simulink model "WBR_Simulator"  (R2023b)
settings: Solver=FixedStepAuto  StartTime=0.0  StopTime=60  FixedStep=0.001  MaxStep=0.001
undefined symbols (not defined in the file or in its folder): DiscIntNeverNeededParam, magnitude, robot_stats, SIMPARAM, X, Y, Z
libraries: sm_lib x73, nesl_utility x50, simulink x17, slpidlib x6, dsparch4 x2
(part 6 of 7)

== system WBR_Simulator/腿建模/并联腿2 ==
  note: 出现过原始角速度跳变的情况
  note: 此处phi0为平行z轴为0,往越往x轴越大
  设定切向力矩 : Inport
  设定径向力 : Inport  Port=2
  Brick Solid : sm_lib/Body Elements/Brick Solid  GraphicAmbientColor=[0.15 0.15 0.15 1.0]  BasedOnType=Mass  BrickDimensions=[SIMPARAM.L5 0.01 0.01]  BrickDimensionsUnits=m  CenterOfMass=[0 0 0]  CenterOfMassUnits=m  GraphicDiffuseColor=[0.2 0.0 0.0]  Density=1000  DensityUnits=kg/m^3  DoExposeReferenceFrame=on  GraphicEmissiveColor=[0.0 0.0 0.0 1.0]  ExportEntireGeometry=on  SerializedFrames=<Frames><Frame><Id>Frame2</Id><Value><Name>A</Name><Origin><Source>GeometricFeature</Source><FeatureName>-x surface</FeatureName></Origin><PrimaryAxis><DefinedDirection>+Y</DefinedDirection><Source>ReferenceFrame</Source><SourceDirection>+Z</SourceDirection><FeatureName></FeatureName></PrimaryAxis><SecondaryAxis><DefinedDirection>+X</DefinedDirection><Source>ReferenceFrame</Source><SourceDirection>+X</SourceDirection><FeatureName></FeatureName></SecondaryAxis></Value></Frame><Frame><Id>Frame3</Id><Value><Name>E</Name><Origin><Source>GeometricFeature</Source><FeatureName>+x surface</FeatureName></Origin><PrimaryAxis><DefinedDirection>+Y</DefinedDirection><Source>ReferenceFrame</Source><SourceDirection>+Z</SourceDirection><FeatureName></FeatureName></PrimaryAxis><SecondaryAxis><DefinedDirection>+X</DefinedDirection><Source>ReferenceFrame</Source><SourceDirection>+X</SourceDirection><FeatureName></FeatureName></SecondaryAxis></Value></Frame></Frames>  MarkerShape=Sphere  MarkerSize=10  GraphicType=FromGeometry  InertiaType=CalculateFromGeometry  Mass=0.00001  MassUnits=kg  MomentsOfInertia=[1 1 1]  MomentsOfInertiaUnits=kg*m^2  GraphicOpacity=1.0  ProductsOfInertia=[0 0 0]  ProductsOfInertiaUnits=kg*m^2  GraphicShininess=75  GraphicSpecularColor=[0.5 0.5 0.5 1.0]  GraphicVisPropType=SimpleVisualProperties
  Brick Solid1 : sm_lib/Body Elements/Brick Solid  GraphicAmbientColor=[0.15 0.15 0.15 1.0]  BasedOnType=Mass  BrickDimensions="[robot_stats.length_thigh  0.01 0.01]"  BrickDimensionsUnits=m  CenterOfMass=[0 0 0]  CenterOfMassUnits=m  GraphicDiffuseColor=[0.0 0.8 1.0]  Density=1000  DensityUnits=kg/m^3  DoExposeReferenceFrame=off  GraphicEmissiveColor=[0.0 0.0 0.0 1.0]  ExportEntireGeometry=off  SerializedFrames=<Frames><Frame><Id>Frame1</Id><Value><Name>A</Name><Origin><Source>GeometricFeature</Source><FeatureName>-x surface</FeatureName></Origin><PrimaryAxis><DefinedDirection>+Y</DefinedDirection><Source>ReferenceFrame</Source><SourceDirection>+Z</SourceDirection><FeatureName></FeatureName></PrimaryAxis><SecondaryAxis><DefinedDirection>+X</DefinedDirection><Source>ReferenceFrame</Source><SourceDirection>+X</SourceDirection><FeatureName></FeatureName></SecondaryAxis></Value></Frame><Frame><Id>Frame2</Id><Value><Name>B</Name><Origin><Source>GeometricFeature</Source><FeatureName>+x surface</FeatureName></Origin><PrimaryAxis><DefinedDirection>-Y</DefinedDirection><Source>ReferenceFrame</Source><SourceDirection>+Z</SourceDirection><FeatureName></FeatureName></PrimaryAxis><SecondaryAxis><DefinedDirection>+X</DefinedDirection><Source>ReferenceFrame</Source><SourceDirection>+X</SourceDirection><FeatureName></FeatureName></SecondaryAxis></Value></Frame></Frames>  MarkerShape=Sphere  MarkerSize=10  GraphicType=FromGeometry  InertiaType=CalculateFromGeometry  Mass=robot_stats.mass_thigh_aver  MassUnits=kg  MomentsOfInertia=[1 1 1]  MomentsOfInertiaUnits=kg*m^2  GraphicOpacity=1.0  ProductsOfInertia=[0 0 0]  ProductsOfInertiaUnits=kg*m^2  GraphicShininess=75  GraphicSpecularColor=[0.5 0.5 0.5 1.0]  GraphicVisPropType=SimpleVisualProperties
  Brick Solid2 : sm_lib/Body Elements/Brick Solid  GraphicAmbientColor=[0.15 0.15 0.15 1.0]  BasedOnType=Mass  BrickDimensions="[robot_stats.length_thigh  0.01 0.01]"  BrickDimensionsUnits=m  CenterOfMass=[0 0 0]  CenterOfMassUnits=m  GraphicDiffuseColor=[0.0 0.8 1.0]  Density=1000  DensityUnits=kg/m^3  DoExposeReferenceFrame=off  GraphicEmissiveColor=[0.0 0.0 0.0 1.0]  ExportEntireGeometry=off  SerializedFrames=<Frames><Frame><Id>Frame1</Id><Value><Name>E</Name><Origin><Source>GeometricFeature</Source><FeatureName>-x surface</FeatureName></Origin><PrimaryAxis><DefinedDirection>-Y</DefinedDirection><Source>ReferenceFrame</Source><SourceDirection>+Z</SourceDirection><FeatureName></FeatureName></PrimaryAxis><SecondaryAxis><DefinedDirection>+X</DefinedDirection><Source>ReferenceFrame</Source><SourceDirection>+X</SourceDirection><FeatureName></FeatureName></SecondaryAxis></Value></Frame><Frame><Id>Frame2</Id><Value><Name>D</Name><Origin><Source>GeometricFeature</Source><FeatureName>+x surface</FeatureName></Origin><PrimaryAxis><DefinedDirection>+Y</DefinedDirection><Source>ReferenceFrame</Source><SourceDirection>+Z</SourceDirection><FeatureName></FeatureName></PrimaryAxis><SecondaryAxis><DefinedDirection>+X</DefinedDirection><Source>ReferenceFrame</Source><SourceDirection>+X</SourceDirection><FeatureName></FeatureName></SecondaryAxis></Value></Frame></Frames>  MarkerShape=Sphere  MarkerSize=10  GraphicType=FromGeometry  InertiaType=CalculateFromGeometry  Mass=robot_stats.mass_thigh_aver  MassUnits=kg  MomentsOfInertia=[1 1 1]  MomentsOfInertiaUnits=kg*m^2  GraphicOpacity=1.0  ProductsOfInertia=[0 0 0]  ProductsOfInertiaUnits=kg*m^2  GraphicShininess=75  GraphicSpecularColor=[0.5 0.5 0.5 1.0]  GraphicVisPropType=SimpleVisualProperties
  Brick Solid3 : sm_lib/Body Elements/Brick Solid  GraphicAmbientColor=[0.15 0.15 0.15 1.0]  BasedOnType=Mass  BrickDimensions="[robot_stats.length_calf  0.01 0.01]"  BrickDimensionsUnits=m  CenterOfMass=[0 0 0]  CenterOfMassUnits=m  GraphicDiffuseColor=[1.0 0.0 0.0]  Density=1000  DensityUnits=kg/m^3  DoExposeReferenceFrame=off  GraphicEmissiveColor=[0.0 0.0 0.0 1.0]  ExportEntireGeometry=off  SerializedFrames=<Frames><Frame><Id>Frame1</Id><Value><Name>B</Name><Origin><Source>GeometricFeature</Source><FeatureName>-x surface</FeatureName></Origin><PrimaryAxis><DefinedDirection>-Y</DefinedDirection><Source>ReferenceFrame</Source><SourceDirection>+Z</SourceDirection><FeatureName></FeatureName></PrimaryAxis><SecondaryAxis><DefinedDirection>+X</DefinedDirection><Source>ReferenceFrame</Source><SourceDirection>+X</SourceDirection><FeatureName></FeatureName></SecondaryAxis></Value></Frame><Frame><Id>Frame2</Id><Value><Name>C</Name><Origin><Source>GeometricFeature</Source><FeatureName>+x surface</FeatureName></Origin><PrimaryAxis><DefinedDirection>-Y</DefinedDirection><Source>ReferenceFrame</Source><SourceDirection>+Z</SourceDirection><FeatureName></FeatureName></PrimaryAxis><SecondaryAxis><DefinedDirection>+X</DefinedDirection><Source>ReferenceFrame</Source><SourceDirection>+X</SourceDirection><FeatureName></FeatureName></SecondaryAxis></Value></Frame></Frames>  MarkerShape=Sphere  MarkerSize=10  GraphicType=FromGeometry  InertiaType=CalculateFromGeometry  Mass=robot_stats.mass_calf_aver  MassUnits=kg  MomentsOfInertia=[1 1 1]  MomentsOfInertiaUnits=kg*m^2  GraphicOpacity=1.0  ProductsOfInertia=[0 0 0]  ProductsOfInertiaUnits=kg*m^2  GraphicShininess=75  GraphicSpecularColor=[0.5 0.5 0.5 1.0]  GraphicVisPropType=SimpleVisualProperties
  Brick Solid4 : sm_lib/Body Elements/Brick Solid  GraphicAmbientColor=[0.15 0.15 0.15 1.0]  BasedOnType=Mass  BrickDimensions="[robot_stats.length_calf  0.01 0.01]"  BrickDimensionsUnits=m  CenterOfMass=[0 0 0]  CenterOfMassUnits=m  GraphicDiffuseColor=[1.0 0.0 0.0]  Density=1000  DensityUnits=kg/m^3  DoExposeReferenceFrame=off  GraphicEmissiveColor=[0.0 0.0 0.0 1.0]  ExportEntireGeometry=off  SerializedFrames=<Frames><Frame><Id>Frame1</Id><Value><Name>C</Name><Origin><Source>GeometricFeature</Source><FeatureName>-x surface</FeatureName></Origin><PrimaryAxis><DefinedDirection>-Y</DefinedDirection><Source>ReferenceFrame</Source><SourceDirection>+Z</SourceDirection><FeatureName></FeatureName></PrimaryAxis><SecondaryAxis><DefinedDirection>+X</DefinedDirection><Source>ReferenceFrame</Source><SourceDirection>+X</SourceDirection><FeatureName></FeatureName></SecondaryAxis></Value></Frame><Frame><Id>Frame2</Id><Value><Name>D</Name><Origin><Source>GeometricFeature</Source><FeatureName>+x surface</FeatureName></Origin><PrimaryAxis><DefinedDirection>-Y</DefinedDirection><Source>ReferenceFrame</Source><SourceDirection>+Z</SourceDirection><FeatureName></FeatureName></PrimaryAxis><SecondaryAxis><DefinedDirection>+X</DefinedDirection><Source>ReferenceFrame</Source><SourceDirection>+X</SourceDirection><FeatureName></FeatureName></SecondaryAxis></Value></Frame></Frames>  MarkerShape=Sphere  MarkerSize=10  GraphicType=FromGeometry  InertiaType=CalculateFromGeometry  Mass=robot_stats.mass_calf_aver  MassUnits=kg  MomentsOfInertia=[1 1 1]  MomentsOfInertiaUnits=kg*m^2  GraphicOpacity=1.0  ProductsOfInertia=[0 0 0]  ProductsOfInertiaUnits=kg*m^2  GraphicShininess=75  GraphicSpecularColor=[0.5 0.5 0.5 1.0]  GraphicVisPropType=SimpleVisualProperties
  Brick Solid5 : sm_lib/Body Elements/Brick Solid  GraphicAmbientColor=[0.15 0.15 0.15 1.0]  BasedOnType=Mass  BrickDimensions=[0.01 0.01 0.01]  BrickDimensionsUnits=m  CenterOfMass=[0 0 0]  CenterOfMassUnits=m  GraphicDiffuseColor=[0.5 0.5 0.5]  Density=1000  DensityUnits=kg/m^3  DoExposeReferenceFrame=on  GraphicEmissiveColor=[0.0 0.0 0.0 1.0]  ExportEntireGeometry=off  SerializedFrames=<Frames><Frame><Id>Frame1</Id><Value><Name>joint</Name><Origin><Source>CenterOfMassFrame</Source><FeatureName></FeatureName></Origin><PrimaryAxis><DefinedDirection>-Z</DefinedDirection><Source>ReferenceFrame</Source><SourceDirection>+Z</SourceDirection><FeatureName></FeatureName></PrimaryAxis><SecondaryAxis><DefinedDirection>+X</DefinedDirection><Source>ReferenceFrame</Source><SourceDirection>+X</SourceDirection><FeatureName></FeatureName></SecondaryAxis></Value></Frame></Frames>  MarkerShape=Sphere  MarkerSize=10  GraphicType=FromGeometry  InertiaType=CalculateFromGeometry  Mass=0.00001  MassUnits=kg  MomentsOfInertia=[1 1 1]  MomentsOfInertiaUnits=kg*m^2  GraphicOpacity=1.0  ProductsOfInertia=[0 0 0]  ProductsOfInertiaUnits=kg*m^2  GraphicShininess=75  GraphicSpecularColor=[0.5 0.5 0.5 1.0]  GraphicVisPropType=SimpleVisualProperties
  Bus Creator : BusCreator  Inputs=4
  Bus Creator1 : BusCreator  Inputs=2
  Bus Creator2 : BusCreator  Inputs=2
  Bus Creator5 : BusCreator  Inputs=2
  Bus Creator6 : BusCreator  Inputs=4
  Bus Selector : BusSelector  OutputSignals=phi_1,phi_4
  Bus Selector1 : BusSelector  OutputSignals=signal2.phi_1,signal2.phi_4,signal2.wphi_1,signal2.wphi_4,signal1.phi_2,signal1.phi_3
  Bus Selector2 : BusSelector  OutputSignals=signal2.phi_1,signal1.phi_2,signal1.phi_3,signal2.phi_4,signal2.wphi_1,signal2.wphi_4
  Connection Label1 : ConnectionLabel  Label=base_frame
  Connection Label6 : ConnectionLabel  Label=base_frame
  PS-Simulink Converter{,1..3} (4 alike) : nesl_utility/PS-Simulink Converter  PhysicalDomain=network_engine_domain  SubClassName=ps_output  LeftPortType=input  RightPortType=output  PseudoPeriodic=off  Frequencies=[]  VectorFormat=1-D array  Unit=inherit  AffineConversion=off
  Revolute Joint : sm_lib/Joints/Revolute Joint  JointMode=Normal  SenseConstraintForce=off  SenseConstraintForceX=off  SenseConstraintForceY=off  SenseConstraintForceZ=off  SenseConstraintTorque=off  SenseConstraintTorqueX=off  SenseConstraintTorqueY=off  SenseConstraintTorqueZ=off  SenseTotalForce=off  SenseTotalForceX=off  SenseTotalForceY=off  SenseTotalForceZ=off  SenseTotalTorque=off  SenseTotalTorqueX=off  SenseTotalTorqueY=off  SenseTotalTorqueZ=off  CompositeWrenchDir=FollowerOnBase  CompositeWrenchFrame=BaseFrame  EquilibriumPosition=0  EquilibriumPositionUnits=deg  SpringStiffness=0  SpringStiffnessUnits=N*m/deg  DampingCoefficient=0  DampingCoefficientUnits=N*m/(deg/s)  TorqueActuationMode=InputTorque  MotionActuationMode=ComputedMotion  SensePosition=on  SenseVelocity=on  SenseAcceleration=off  SenseTorqueForce=off  SenseLowerLimitTorqueForce=off  SenseUpperLimitTorqueForce=off  LowerLimitSpecify=off  LowerLimitBound=-90  LowerLimitBoundUnits=deg  LowerLimitStiffness=1e4  LowerLimitStiffnessUnits=N*m/deg  LowerLimitDamping=10  LowerLimitDampingUnits=N*m/(deg/s)  LowerLimitTransitionRegionWidth=0.1  LowerLimitTransitionRegionWidthUnits=deg  UpperLimitSpecify=off  UpperLimitBound=90  UpperLimitBoundUnits=deg  UpperLimitStiffness=1e4  UpperLimitStiffnessUnits=N*m/deg  UpperLimitDamping=10  UpperLimitDampingUnits=N*m/(deg/s)  UpperLimitTransitionRegionWidth=0.1  UpperLimitTransitionRegionWidthUnits=deg  PositionTargetSpecify=on  PositionTargetPriority=High  PositionTargetValue=SIMPARAM.init_phi1  PositionTargetValueUnits=rad  VelocityTargetSpecify=off  VelocityTargetPriority=High  VelocityTargetValue=0  VelocityTargetValueUnits=deg/s
  Revolute Joint1 : sm_lib/Joints/Revolute Joint  JointMode=Normal  SenseConstraintForce=off  SenseConstraintForceX=off  SenseConstraintForceY=off  SenseConstraintForceZ=off  SenseConstraintTorque=off  SenseConstraintTorqueX=off  SenseConstraintTorqueY=off  SenseConstraintTorqueZ=off  SenseTotalForce=off  SenseTotalForceX=off  SenseTotalForceY=off  SenseTotalForceZ=off  SenseTotalTorque=off  SenseTotalTorqueX=off  SenseTotalTorqueY=off  SenseTotalTorqueZ=off  CompositeWrenchDir=FollowerOnBase  CompositeWrenchFrame=BaseFrame  EquilibriumPosition=0  EquilibriumPositionUnits=deg  SpringStiffness=0  SpringStiffnessUnits=N*m/deg  DampingCoefficient=0  DampingCoefficientUnits=N*m/(deg/s)  TorqueActuationMode=InputTorque  MotionActuationMode=ComputedMotion  SensePosition=on  SenseVelocity=on  SenseAcceleration=off  SenseTorqueForce=off  SenseLowerLimitTorqueForce=off  SenseUpperLimitTorqueForce=off  LowerLimitSpecify=off  LowerLimitBound=-90  LowerLimitBoundUnits=deg  LowerLimitStiffness=1e4  LowerLimitStiffnessUnits=N*m/deg  LowerLimitDamping=10  LowerLimitDampingUnits=N*m/(deg/s)  LowerLimitTransitionRegionWidth=0.1  LowerLimitTransitionRegionWidthUnits=deg  UpperLimitSpecify=off  UpperLimitBound=90  UpperLimitBoundUnits=deg  UpperLimitStiffness=1e4  UpperLimitStiffnessUnits=N*m/deg  UpperLimitDamping=10  UpperLimitDampingUnits=N*m/(deg/s)  UpperLimitTransitionRegionWidth=0.1  UpperLimitTransitionRegionWidthUnits=deg  PositionTargetSpecify=on  PositionTargetPriority=High  PositionTargetValue=SIMPARAM.init_phi4  PositionTargetValueUnits=rad  VelocityTargetSpecify=off  VelocityTargetPriority=High  VelocityTargetValue=0  VelocityTargetValueUnits=deg/s
  Revolute Joint2 : sm_lib/Joints/Revolute Joint  JointMode=Normal  SenseConstraintForce=off  SenseConstraintForceX=off  SenseConstraintForceY=off  SenseConstraintForceZ=off  SenseConstraintTorque=off  SenseConstraintTorqueX=off  SenseConstraintTorqueY=off  SenseConstraintTorqueZ=off  SenseTotalForce=off  SenseTotalForceX=off  SenseTotalForceY=off  SenseTotalForceZ=off  SenseTotalTorque=off  SenseTotalTorqueX=off  SenseTotalTorqueY=off  SenseTotalTorqueZ=off  CompositeWrenchDir=FollowerOnBase  CompositeWrenchFrame=BaseFrame  EquilibriumPosition=0  EquilibriumPositionUnits=deg  SpringStiffness=0  SpringStiffnessUnits=N*m/deg  DampingCoefficient=0  DampingCoefficientUnits=N*m/(deg/s)  TorqueActuationMode=NoTorque  MotionActuationMode=ComputedMotion  SensePosition=off  SenseVelocity=off  SenseAcceleration=off  SenseTorqueForce=off  SenseLowerLimitTorqueForce=off  SenseUpperLimitTorqueForce=off  LowerLimitSpecify=off  LowerLimitBound=-90  LowerLimitBoundUnits=deg  LowerLimitStiffness=1e4  LowerLimitStiffnessUnits=N*m/deg  LowerLimitDamping=10  LowerLimitDampingUnits=N*m/(deg/s)  LowerLimitTransitionRegionWidth=0.1  LowerLimitTransitionRegionWidthUnits=deg  UpperLimitSpecify=off  UpperLimitBound=90  UpperLimitBoundUnits=deg  UpperLimitStiffness=1e4  UpperLimitStiffnessUnits=N*m/deg  UpperLimitDamping=10  UpperLimitDampingUnits=N*m/(deg/s)  UpperLimitTransitionRegionWidth=0.1  UpperLimitTransitionRegionWidthUnits=deg  PositionTargetSpecify=on  PositionTargetPriority=High  PositionTargetValue=SIMPARAM.init_phi1-SIMPARAM.init_phi2  PositionTargetValueUnits=rad  VelocityTargetSpecify=off  VelocityTargetPriority=High  VelocityTargetValue=0  VelocityTargetValueUnits=deg/s
  Revolute Joint3 : sm_lib/Joints/Revolute Joint  JointMode=Normal  SenseConstraintForce=off  SenseConstraintForceX=off  SenseConstraintForceY=off  SenseConstraintForceZ=off  SenseConstraintTorque=off  SenseConstraintTorqueX=off  SenseConstraintTorqueY=off  SenseConstraintTorqueZ=off  SenseTotalForce=off  SenseTotalForceX=off  SenseTotalForceY=off  SenseTotalForceZ=off  SenseTotalTorque=off  SenseTotalTorqueX=off  SenseTotalTorqueY=off  SenseTotalTorqueZ=off  CompositeWrenchDir=FollowerOnBase  CompositeWrenchFrame=BaseFrame  EquilibriumPosition=0  EquilibriumPositionUnits=deg  SpringStiffness=0  SpringStiffnessUnits=N*m/deg  DampingCoefficient=0  DampingCoefficientUnits=N*m/(deg/s)  TorqueActuationMode=NoTorque  MotionActuationMode=ComputedMotion  SensePosition=off  SenseVelocity=off  SenseAcceleration=off  SenseTorqueForce=off  SenseLowerLimitTorqueForce=off  SenseUpperLimitTorqueForce=off  LowerLimitSpecify=off  LowerLimitBound=-90  LowerLimitBoundUnits=deg  LowerLimitStiffness=1e4  LowerLimitStiffnessUnits=N*m/deg  LowerLimitDamping=10  LowerLimitDampingUnits=N*m/(deg/s)  LowerLimitTransitionRegionWidth=0.1  LowerLimitTransitionRegionWidthUnits=deg  UpperLimitSpecify=off  UpperLimitBound=90  UpperLimitBoundUnits=deg  UpperLimitStiffness=1e4  UpperLimitStiffnessUnits=N*m/deg  UpperLimitDamping=10  UpperLimitDampingUnits=N*m/(deg/s)  UpperLimitTransitionRegionWidth=0.1  UpperLimitTransitionRegionWidthUnits=deg  PositionTargetSpecify=on  PositionTargetPriority=High  PositionTargetValue=pi-(SIMPARAM.init_phi3-SIMPARAM.init_phi4)  PositionTargetValueUnits=rad  VelocityTargetSpecify=off  VelocityTargetPriority=High  VelocityTargetValue=0  VelocityTargetValueUnits=deg/s
  Revolute Joint5 : sm_lib/Joints/Revolute Joint  JointMode=Normal  SenseConstraintForce=off  SenseConstraintForceX=off  SenseConstraintForceY=off  SenseConstraintForceZ=off  SenseConstraintTorque=off  SenseConstraintTorqueX=off  SenseConstraintTorqueY=off  SenseConstraintTorqueZ=off  SenseTotalForce=off  SenseTotalForceX=off  SenseTotalForceY=off  SenseTotalForceZ=off  SenseTotalTorque=off  SenseTotalTorqueX=off  SenseTotalTorqueY=off  SenseTotalTorqueZ=off  CompositeWrenchDir=FollowerOnBase  CompositeWrenchFrame=BaseFrame  EquilibriumPosition=0  EquilibriumPositionUnits=deg  SpringStiffness=0  SpringStiffnessUnits=N*m/deg  DampingCoefficient=0  DampingCoefficientUnits=N*m/(deg/s)  TorqueActuationMode=NoTorque  MotionActuationMode=ComputedMotion  SensePosition=off  SenseVelocity=off  SenseAcceleration=off  SenseTorqueForce=off  SenseLowerLimitTorqueForce=off  SenseUpperLimitTorqueForce=off  LowerLimitSpecify=off  LowerLimitBound=-90  LowerLimitBoundUnits=deg  LowerLimitStiffness=1e4  LowerLimitStiffnessUnits=N*m/deg  LowerLimitDamping=10  LowerLimitDampingUnits=N*m/(deg/s)  LowerLimitTransitionRegionWidth=0.1  LowerLimitTransitionRegionWidthUnits=deg  UpperLimitSpecify=off  UpperLimitBound=90  UpperLimitBoundUnits=deg  UpperLimitStiffness=1e4  UpperLimitStiffnessUnits=N*m/deg  UpperLimitDamping=10  UpperLimitDampingUnits=N*m/(deg/s)  UpperLimitTransitionRegionWidth=0.1  UpperLimitTransitionRegionWidthUnits=deg  PositionTargetSpecify=off  PositionTargetPriority=High  PositionTargetValue=0  PositionTargetValueUnits=deg  VelocityTargetSpecify=off  VelocityTargetPriority=High  VelocityTargetValue=0  VelocityTargetValueUnits=deg/s
  Simulink-PS Converter : nesl_utility/Simulink-PS Converter  PhysicalDomain=network_engine_domain  SubClassName=ps_input  LeftPortType=input  RightPortType=output  PseudoPeriodic=off  Frequencies=[]  NoiseDistribution=none  NoiseParameters=[]  Unit=1  AffineConversion=off  FilteringAndDerivatives=provide  SimscapeFilterOrder=1  InputFilterTimeConstant=0.001  UdotUserProvided=0
  Simulink-PS Converter1 : nesl_utility/Simulink-PS Converter  PhysicalDomain=network_engine_domain  SubClassName=ps_input  LeftPortType=input  RightPortType=output  PseudoPeriodic=off  Frequencies=[]  NoiseDistribution=none  NoiseParameters=[]  Unit=1  AffineConversion=off  FilteringAndDerivatives=provide  SimscapeFilterOrder=1  InputFilterTimeConstant=0.001  UdotUserProvided=0
  Spatial Contact Force2 : sm_lib/Forces and Torques/Spatial Contact Force  SenseContactBaseRotation=off  SenseContactBaseTranslation=off  CoefficientOfDynamicFriction=0.3  CoefficientOfStaticFriction=0.5  NormalDamping=1e6  NormalDampingUnits=N/(m/s)  SenseContactSignal=off  NormalStiffness=1e6  NormalStiffnessUnits=N/m  FrictionalCriticalVelocity=1e-3  FrictionalCriticalVelocityUnits=m/s  ZeroCrossDetectContactStartAndEnd=off  SenseContactFollowerRotation=off  SenseContactFollowerTranslation=off  FrictionType=SmoothStickSlip  SenseFrictionalForceMagnitude=off  SenseNormalForceMagnitude=off  NormalForceType=SmoothSpringDamper  SenseNormalVelocity=off  SensePenetrationDepth=off  SenseSeparationDistance=off  SenseTangentialVelocity=off  NormalTransitionRegionWidth=1e-4  NormalTransitionRegionWidthUnits=m
  Spatial Contact Force7 : sm_lib/Forces and Torques/Spatial Contact Force  SenseContactBaseRotation=off  SenseContactBaseTranslation=off  CoefficientOfDynamicFriction=0.3  CoefficientOfStaticFriction=0.5  NormalDamping=1e6  NormalDampingUnits=N/(m/s)  SenseContactSignal=off  NormalStiffness=1e6  NormalStiffnessUnits=N/m  FrictionalCriticalVelocity=1e-3  FrictionalCriticalVelocityUnits=m/s  ZeroCrossDetectContactStartAndEnd=off  SenseContactFollowerRotation=off  SenseContactFollowerTranslation=off  FrictionType=SmoothStickSlip  SenseFrictionalForceMagnitude=off  SenseNormalForceMagnitude=off  NormalForceType=SmoothSpringDamper  SenseNormalVelocity=off  SensePenetrationDepth=off  SenseSeparationDistance=off  SenseTangentialVelocity=off  NormalTransitionRegionWidth=1e-4  NormalTransitionRegionWidthUnits=m
  Zero-Order Hold{,1..3} (4 alike) : ZeroOrderHold  SampleTime=0.001
  五连杆正解算矩阵(关节转至末端) : Subsystem
  腿末端控制器 : Subsystem
  解算phi2&phi3_1 : Subsystem
  运动学解算验证(仅可证明旋转矩阵 : Subsystem
  基坐标 : PMIOPort  Side=Left
  轮毂坐标轴 : PMIOPort  Port=2  Side=Left
  底盘地面碰撞 : PMIOPort  Port=3  Side=Right
  底盘飞坡碰撞 : PMIOPort  Port=4  Side=Right
  phi_0 : Outport
  L_0 : Outport  Port=2
  real_vq : Outport  Port=3
  real_vd : Outport  Port=4
  valid_tqd : Outport  Port=5
  wires:
  Bus Creator2/1 -> Bus Selector2/1, Bus Selector1/1  "腿关节角度集"
  腿末端控制器/3(R) -> [R]
  Bus Selector1/2 -> 五连杆正解算矩阵(关节转至末端)/2(phi_4)  "<phi_4>"
  Bus Creator/1 -> Bus Creator2/2, Bus Selector/1
  Bus Selector1/6 -> 五连杆正解算矩阵(关节转至末端)/6(phi_3)  "<phi_3>"
  五连杆正解算矩阵(关节转至末端)/1(J) -> 腿末端控制器/6(J)  "J矩阵"
  Bus Selector/1 -> 解算phi2&phi3_1/1(phi1)  "<phi_1>"
  Bus Selector2/2 -> Bus Creator6/2  "<phi_2>"
  Bus Selector/2 -> 解算phi2&phi3_1/2(phi4)  "<phi_4>"
  腿末端控制器/4(R_inv) -> [R_inv]
  Bus Selector1/4 -> 五连杆正解算矩阵(关节转至末端)/4(wphi_4)  "<wphi_4>"
  Bus Selector1/3 -> 五连杆正解算矩阵(关节转至末端)/3(wphi_1)  "<wphi_1>"
  Bus Selector1/5 -> 五连杆正解算矩阵(关节转至末端)/5(phi_2)  "<phi_2>"
  Bus Selector2/5 -> 腿末端控制器/2(wphi_1)  "<wphi_1>"
  Bus Selector2/6 -> 腿末端控制器/3(wphi_4)  "<wphi_4>"
  Bus Selector1/1 -> 五连杆正解算矩阵(关节转至末端)/1(phi_1)  "<phi_1>"
  [R_inv] -> 运动学解算验证(仅可证明旋转矩阵/2(R_inv)
  [R] -> 运动学解算验证(仅可证明旋转矩阵/1(R)
  Bus Creator1/1 -> ?  "关节扭矩"
  腿末端控制器/5(phi_0) -> phi_0/1
  腿末端控制器/6(L_0) -> L_0/1
  腿末端控制器/8(real_vd) -> real_vd/1
  腿末端控制器/7(real_vq) -> real_vq/1
  设定切向力矩/1 -> 腿末端控制器/4(set_tq)
  设定径向力/1 -> 腿末端控制器/5(set_fd)
  PS-Simulink Converter/1 -> Zero-Order Hold/1
  PS-Simulink Converter1/1 -> Zero-Order Hold1/1
  腿末端控制器/1(torque_1) -> Bus Creator1/1, Simulink-PS Converter/1
  腿末端控制器/2(torque_4) -> Bus Creator1/2, Simulink-PS Converter1/1
  PS-Simulink Converter2/1 -> Zero-Order Hold2/1
  PS-Simulink Converter3/1 -> Zero-Order Hold3/1
  腿末端控制器/9(valid_tqd) -> valid_tqd/1
  解算phi2&phi3_1/1(phi2) -> Bus Creator5/1  "phi_2"
  解算phi2&phi3_1/2(phi3) -> Bus Creator5/2  "phi_3"
  Bus Creator5/1 -> Bus Creator2/1
  Bus Selector2/1 -> Bus Creator6/1  "<phi_1>"
  Bus Selector2/4 -> Bus Creator6/4  "<phi_4>"
  Bus Selector2/3 -> Bus Creator6/3  "<phi_3>"
  Bus Creator6/1 -> 腿末端控制器/1(phi)
  Zero-Order Hold/1 -> Bus Creator/1  "phi_1"
  Zero-Order Hold1/1 -> Bus Creator/2  "phi_4"
  Zero-Order Hold2/1 -> Bus Creator/3  "wphi_1"
  Zero-Order Hold3/1 -> Bus Creator/4  "wphi_4"
  connections:
  Brick Solid/LConn2 -- Revolute Joint1/LConn1
  Revolute Joint2/RConn1 -- Brick Solid3/LConn1
  PS-Simulink Converter1/LConn1 -- Revolute Joint1/RConn2
  Revolute Joint/LConn1 -- Brick Solid/LConn1
  Revolute Joint/RConn2 -- PS-Simulink Converter/LConn1
  Brick Solid4/RConn1 -- Revolute Joint3/RConn1
  Revolute Joint/RConn1 -- Brick Solid1/LConn1
  Brick Solid4/LConn1 -- Revolute Joint5/LConn1
  Brick Solid5/RConn1 -- Brick Solid3/RConn1 -- Revolute Joint5/RConn1 -- 运动学解算验证(仅可证明旋转矩阵/RConn1
  Revolute Joint/RConn3 -- PS-Simulink Converter2/LConn1
  Connection Label6/LConn1 -- 运动学解算验证(仅可证明旋转矩阵/LConn1
  Revolute Joint1/RConn3 -- PS-Simulink Converter3/LConn1
  Brick Solid2/RConn1 -- Revolute Joint3/LConn1
  基坐标/RConn1 -- Connection Label1/LConn1 -- Brick Solid/RConn1
  Revolute Joint/LConn2 -- Simulink-PS Converter/RConn1
  Simulink-PS Converter1/RConn1 -- Revolute Joint1/LConn2
  Revolute Joint1/RConn1 -- Brick Solid2/LConn1
  Brick Solid5/LConn1 -- 轮毂坐标轴/RConn1
  Brick Solid1/RConn1 -- Revolute Joint2/LConn1
  Spatial Contact Force2/LConn1 -- 底盘地面碰撞/RConn1
  Spatial Contact Force7/RConn1 -- Brick Solid/RConn2 -- Spatial Contact Force2/RConn1
  Spatial Contact Force7/LConn1 -- 底盘飞坡碰撞/RConn1

== system WBR_Simulator/腿建模/串联腿/五连杆正解算矩阵(关节转至末端) ==
  phi_1 : Inport
  phi_2 : Inport  Port=2
  Add : Sum  Inputs=-+
  Add1 : Sum  Inputs=-+
  Add2 : Sum  Inputs=+-
  Add3 : Sum  Inputs=+-
  Constant : Constant  Value=SIMPARAM.L2
  Constant1 : Constant  Value=SIMPARAM.L2
  Constant{2,4..5,7} (4 alike) : Constant  Value=0
  Constant3 : Constant  Value=SIMPARAM.L1
  Constant8 : Constant  Value=SIMPARAM.L1
  Divide{,1..3} (4 alike) : Product  Inputs=**
  MATLAB Function : MATLAB Function  TreatAsAtomicUnit=on
  Sin1 : Trigonometry
  Sin2 : Trigonometry
  Sin3 : Trigonometry  Operator=cos
  Sin4 : Trigonometry  Operator=cos
  J : Outport
  wires:
  phi_1/1 -> [phi_1]
  phi_2/1 -> [phi_2]
  [phi_1] -> Sin1/1
  MATLAB Function/1(J) -> J/1
  Constant4/1 -> Add/2
  Sin1/1 -> Add/1
  Constant8/1 -> Divide/2
  Add/1 -> Divide/1
  Add1/1 -> Divide1/1
  Sin2/1 -> Add1/1
  Constant2/1 -> Add1/2
  [phi_2] -> Sin2/1
  Constant/1 -> Divide1/2
  Add2/1 -> Divide2/1
  Sin3/1 -> Add2/1
  Constant5/1 -> Add2/2
  [phi_1] -> Sin3/1
  Constant3/1 -> Divide2/2
  Constant1/1 -> Divide3/2
  Constant7/1 -> Add3/2
  Add3/1 -> Divide3/1
  [phi_2] -> Sin4/1
  Sin4/1 -> Add3/1
  Divide/1 -> MATLAB Function/1(J11)
  Divide1/1 -> MATLAB Function/2(J12)
  Divide2/1 -> MATLAB Function/3(J21)
  Divide3/1 -> MATLAB Function/4(J22)

== system WBR_Simulator/腿建模/串联腿/腿末端控制器 ==
  phi : Inport
  wphi_1 : Inport  Port=2
  wphi_2 : Inport  Port=3
  set_tq : Inport  Port=4
  set_fd : Inport  Port=5
  J : Inport  Port=6
  Bus Selector : BusSelector  OutputSignals=phi_1,phi_2
  Constant : Constant  Value=0
  Constant1 : Constant
  Constant2 : Constant
  Constant3 : Constant  Value=0
  Divide : Product  Inputs=*/
  From2 : From  Commented=on  GotoTag=real_vxy
  From5 : From  Commented=on  GotoTag=J
  Mux : Mux  Inputs=2
  Mux1 : Mux
  Product : Product  Inputs=/  Multiplication=Matrix(*)
  Product8 : Product  Multiplication=Matrix(*)
  Reshape : Reshape  OutputDimensionality=Customize  OutputDimensions=[2,2]
  xy运动 : Subsystem  Commented=on
  极坐标运动控制器 : Subsystem
  笛卡尔坐标系转极坐标系 : Subsystem
  torque_1 : Outport
  torque_2 : Outport  Port=2
  R : Outport  Port=3
  R_inv : Outport  Port=4
  phi_0 : Outport  Port=5
  L_0 : Outport  Port=6
  real_vq : Outport  Port=7
  real_vd : Outport  Port=8
  valid_tqd : Outport  Port=9
  wires:
  J/1 -> [J]
  wphi_1/1 -> [wphi_1]
  wphi_2/1 -> [wphi_2]
  Product8/1 -> [real_vxy]
  [wphi_2] -> Mux/2
  [J] -> Product8/1
  Mux/1 -> Product8/2
  [wphi_1] -> Mux/1
  From2/1 -> xy运动/1(real_vxy)
  [real_vxy] -> 极坐标运动控制器/1(real_vxy)
  [R] -> 极坐标运动控制器/2(R)
  [J] -> 极坐标运动控制器/3(J)
  From5/1 -> xy运动/2(J)
  笛卡尔坐标系转极坐标系/1(R) -> [R], R/1, Product/1
  Product/1 -> R_inv/1
  极坐标运动控制器/2(torque_2) -> torque_2/1
  极坐标运动控制器/1(torque_1) -> torque_1/1
  笛卡尔坐标系转极坐标系/3(L_0) -> [L_0], L_0/1
  笛卡尔坐标系转极坐标系/2(phi_0) -> phi_0/1
  set_tq/1 -> 极坐标运动控制器/6(set_tq)
  set_fd/1 -> 极坐标运动控制器/7(set_fd)
  极坐标运动控制器/4(real_vd) -> real_vd/1
  极坐标运动控制器/3(real_vq) -> real_vq/1
  [phi_2] -> 笛卡尔坐标系转极坐标系/2(phi_2)
  [phi_1] -> 笛卡尔坐标系转极坐标系/1(phi_1)
  Mux1/1 -> Reshape/1
  [L_0] -> Divide/2
  Constant1/1 -> Mux1/4  "M22"
  Reshape/1 -> [M]
  [M] -> 极坐标运动控制器/4(M)
  Constant/1 -> Mux1/3  "M12"
  Constant3/1 -> Mux1/2  "M21"
  Constant2/1 -> Divide/1
  Divide/1 -> Mux1/1  "M11"
  极坐标运动控制器/5(valid_tqd) -> valid_tqd/1
  [phi] -> 极坐标运动控制器/5(In5)
  Bus Selector/1 -> [phi_1]  "<phi_1>"
  Bus Selector/2 -> [phi_2]  "<phi_2>"
  phi/1 -> [phi], Bus Selector/1

== system WBR_Simulator/腿建模/串联腿/运动学解算验证(仅可证明旋转矩阵 ==
  R : Inport
  R_inv : Inport  Port=2
  Bus Creator1 : BusCreator  Inputs=2
  Bus Creator3 : BusCreator  Inputs=2
  Discrete Derivative : simulink/Discrete/Discrete Derivative  gainval=1.0  ICPrevScaledInput=0.0  OutMin=[]  OutMax=[]  OutDataType=fixdt(1, 16)  OutScaling=2^-10  DoSatur=off
  Discrete Derivative1 : simulink/Discrete/Discrete Derivative  gainval=1.0  ICPrevScaledInput=0.0  OutMin=[]  OutMax=[]  OutDataType=fixdt(1, 16)  OutScaling=2^-10  DoSatur=off
  Mux : Mux  Inputs=2
  Mux1 : Mux  Inputs=2
  PS-Simulink Converter{4..7} (4 alike) : nesl_utility/PS-Simulink Converter  PhysicalDomain=network_engine_domain  SubClassName=ps_output  LeftPortType=input  RightPortType=output  PseudoPeriodic=off  Frequencies=[]  VectorFormat=1-D array  Unit=inherit  AffineConversion=off
  Product : Product
  Product1 : Product  Multiplication=Matrix(*)
  Product2 : Product  Multiplication=Matrix(*)
  Transform Sensor : sm_lib/Frames and Transforms/Transform Sensor  MeasurementFrame=Base  RotationSequence=XYX  SenseAngle=off  SenseAxis=off  SenseQ=off  SenseR=off  SenseRotationSequence=off  SenseOmegaX=off  SenseOmegaY=off  SenseOmegaZ=off  SenseOmega=off  SenseQDot=off  SenseRDot=off  SenseRotationSequenceDot=off  SenseAlphaX=off  SenseAlphaY=off  SenseAlphaZ=off  SenseAlpha=off  SenseQDDot=off  SenseRDDot=off  SenseX=on  SenseY=off  SenseZ=on  SenseXYZ=off  SenseRad=off  SenseAzim=off  SenseDist=off  SenseInc=off  SenseXDot=on  SenseYDot=off  SenseZDot=on  SenseXYZDot=off  SenseRadDot=off  SenseAzimDot=off  SenseDistDot=off  SenseIncDot=off  SenseXDDot=off  SenseYDDot=off  SenseZDDot=off  SenseXYZDDot=off  SenseRadDDot=off  SenseAzimDDot=off  SenseDistDDot=off  SenseIncDDot=off
  Zero-Order Hold{,1..3} (4 alike) : ZeroOrderHold  SampleTime=0.001
  笛卡尔转极坐标 : Subsystem
  五连杆末端坐标 : PMIOPort  Side=Right
  基坐标 : PMIOPort  Port=2  Side=Left
  wires:
  PS-Simulink Converter6/1 -> Zero-Order Hold2/1  "vx"
  Discrete Derivative/1 -> Product/1
  Product1/1 -> ?  "代算C点正交坐标速度"
  [R] -> Product2/1
  Discrete Derivative1/1 -> Mux/2, Bus Creator1/2  "vd"
  笛卡尔转极坐标/2(L_0) -> Discrete Derivative1/1, Product/2
  Mux/1 -> Product1/2
  笛卡尔转极坐标/1(phi_0) -> Discrete Derivative/1
  [R_inv] -> Product1/1
  Product/1 -> Mux/1, Bus Creator1/1  "vq"
  PS-Simulink Converter5/1 -> Zero-Order Hold1/1
  Bus Creator1/1 -> ?  "真实C点极坐标速度"
  PS-Simulink Converter4/1 -> Zero-Order Hold/1
  Mux1/1 -> Product2/2
  Product2/1 -> ?  "代算C点极坐标速度"
  Bus Creator3/1 -> ?  "真实C点正交坐标速度"
  R/1 -> [R]
  R_inv/1 -> [R_inv]
  Zero-Order Hold/1 -> 笛卡尔转极坐标/1(x)
  Zero-Order Hold1/1 -> 笛卡尔转极坐标/2(z)
  Zero-Order Hold2/1 -> Mux1/1, Bus Creator3/1
  PS-Simulink Converter7/1 -> Zero-Order Hold3/1  "vz"
  Zero-Order Hold3/1 -> Mux1/2, Bus Creator3/2
  connections:
  PS-Simulink Converter5/LConn1 -- Transform Sensor/RConn3
  PS-Simulink Converter4/LConn1 -- Transform Sensor/RConn2
  Transform Sensor/RConn1 -- 五连杆末端坐标/RConn1
  基坐标/RConn1 -- Transform Sensor/LConn1
  PS-Simulink Converter6/LConn1 -- Transform Sensor/RConn4
  PS-Simulink Converter7/LConn1 -- Transform Sensor/RConn5

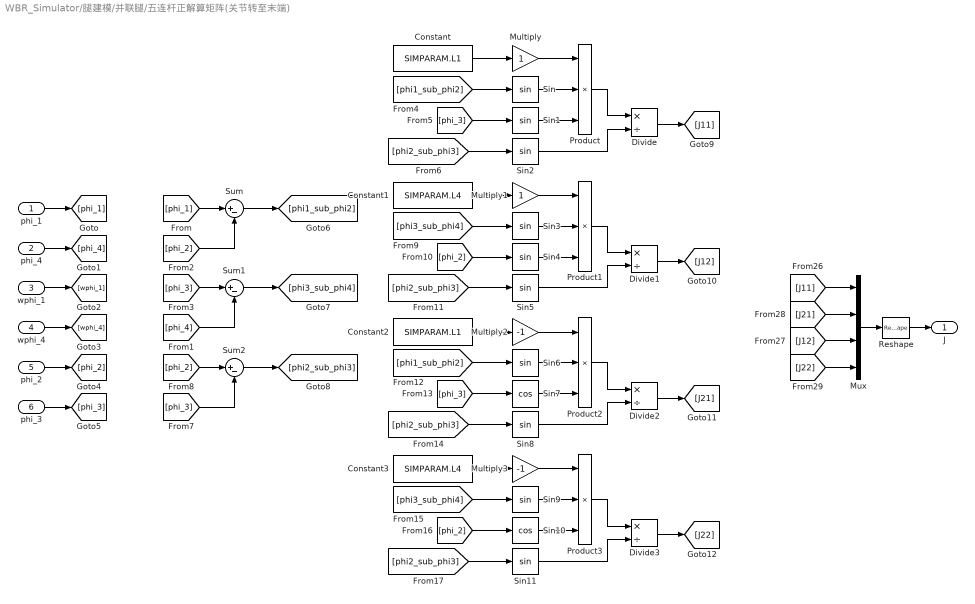
== system WBR_Simulator/腿建模/并联腿/五连杆正解算矩阵(关节转至末端) ==
  phi_1 : Inport
  phi_4 : Inport  Port=2
  wphi_1 : Inport  Port=3
  wphi_4 : Inport  Port=4
  phi_2 : Inport  Port=5
  phi_3 : Inport  Port=6
  Constant : Constant  Value=SIMPARAM.L1
  Constant1 : Constant  Value=SIMPARAM.L4
  Constant2 : Constant  Value=SIMPARAM.L1
  Constant3 : Constant  Value=SIMPARAM.L4
  Divide{,1..3} (4 alike) : Product  Inputs=*/
  Multiply : Gain
  Multiply1 : Gain
  Multiply2 : Gain  Gain=-1
  Multiply3 : Gain  Gain=-1
  Mux : Mux
  Product{,1..3} (4 alike) : Product  Inputs=3
  Reshape : Reshape  OutputDimensionality=Customize  OutputDimensions=[2,2]
  Sin{,1..6,8..9,11} (10 alike) : Trigonometry
  Sin10 : Trigonometry  Operator=cos
  Sin7 : Trigonometry  Operator=cos
  Sum : Sum  Inputs=|+-
  Sum1 : Sum  Inputs=|+-
  Sum2 : Sum  Inputs=|+-
  J : Outport
  wires:
  phi_1/1 -> [phi_1]
  phi_4/1 -> [phi_4]
  wphi_1/1 -> [wphi_1]
  wphi_4/1 -> [wphi_4]
  phi_2/1 -> [phi_2]
  phi_3/1 -> [phi_3]
  [phi_1] -> Sum/1
  [phi_2] -> Sum/2
  Sum/1 -> [phi1_sub_phi2]
  Sum1/1 -> [phi3_sub_phi4]
  [phi_3] -> Sum1/1
  [phi_4] -> Sum1/2
  [phi1_sub_phi2] -> Sin/1
  Sin/1 -> Product/2
  Constant/1 -> Multiply/1
  Multiply/1 -> Product/1
  [phi_3] -> Sin1/1
  Sin1/1 -> Product/3
  Product/1 -> Divide/1
  [phi2_sub_phi3] -> Sin2/1
  Sin2/1 -> Divide/2
  [phi_3] -> Sum2/2
  [phi_2] -> Sum2/1
  Sum2/1 -> [phi2_sub_phi3]
  Divide/1 -> [J11]
  Product1/1 -> Divide1/1
  Constant1/1 -> Multiply1/1
  [phi3_sub_phi4] -> Sin3/1
  Divide1/1 -> [J12]
  Sin5/1 -> Divide1/2
  [phi_2] -> Sin4/1
  Multiply1/1 -> Product1/1
  Sin4/1 -> Product1/3
  [phi2_sub_phi3] -> Sin5/1
  Sin3/1 -> Product1/2
  Product2/1 -> Divide2/1
  Constant2/1 -> Multiply2/1
  [phi1_sub_phi2] -> Sin6/1
  Divide2/1 -> [J21]
  Sin8/1 -> Divide2/2
  [phi_3] -> Sin7/1
  Multiply2/1 -> Product2/1
  Sin7/1 -> Product2/3
  [phi2_sub_phi3] -> Sin8/1
  Sin6/1 -> Product2/2
  Product3/1 -> Divide3/1
  Constant3/1 -> Multiply3/1
  [phi3_sub_phi4] -> Sin9/1
  Divide3/1 -> [J22]
  Sin11/1 -> Divide3/2
  [phi_2] -> Sin10/1
  Multiply3/1 -> Product3/1
  Sin10/1 -> Product3/3
  [phi2_sub_phi3] -> Sin11/1
  Sin9/1 -> Product3/2
  [J11] -> Mux/1
  [J22] -> Mux/4
  Mux/1 -> Reshape/1
  Reshape/1 -> J/1
  [J21] -> Mux/2
  [J12] -> Mux/3

== system WBR_Simulator/腿建模/并联腿/腿末端控制器 ==
  phi : Inport
  wphi_1 : Inport  Port=2
  wphi_4 : Inport  Port=3
  set_tq : Inport  Port=4
  set_fd : Inport  Port=5
  J : Inport  Port=6
  Bus Selector : BusSelector  OutputSignals=phi_1,phi_2
  Constant : Constant  Value=0
  Constant1 : Constant
  Constant2 : Constant
  Constant3 : Constant  Value=0
  Divide : Product  Inputs=*/
  Mux : Mux  Inputs=2
  Mux1 : Mux
  Product : Product  Inputs=/  Multiplication=Matrix(*)
  Product8 : Product  Multiplication=Matrix(*)
  Reshape : Reshape  OutputDimensionality=Customize  OutputDimensions=[2,2]
  极坐标运动控制器 : Subsystem
  笛卡尔坐标系转极坐标系 : Subsystem
  torque_1 : Outport
  torque_4 : Outport  Port=2
  R : Outport  Port=3
  R_inv : Outport  Port=4
  phi_0 : Outport  Port=5
  L_0 : Outport  Port=6
  real_vq : Outport  Port=7
  real_vd : Outport  Port=8
  valid_tqd : Outport  Port=9
  wires:
  J/1 -> [J]
  wphi_1/1 -> [wphi_1]
  wphi_4/1 -> [wphi_4]
  Product8/1 -> [real_vxy]
  [wphi_4] -> Mux/2
  [J] -> Product8/1
  Mux/1 -> Product8/2
  [wphi_1] -> Mux/1
  [real_vxy] -> 极坐标运动控制器/1(real_vxy)
  [R] -> 极坐标运动控制器/2(R)
  [J] -> 极坐标运动控制器/3(J)
  笛卡尔坐标系转极坐标系/1(R) -> [R], R/1, Product/1
  Product/1 -> R_inv/1
  极坐标运动控制器/2(torque_4) -> torque_4/1
  极坐标运动控制器/1(torque_1) -> torque_1/1
  笛卡尔坐标系转极坐标系/3(L_0) -> [L_0], L_0/1
  笛卡尔坐标系转极坐标系/2(phi_0) -> phi_0/1
  set_tq/1 -> 极坐标运动控制器/6(set_tq)
  set_fd/1 -> 极坐标运动控制器/7(set_fd)
  极坐标运动控制器/4(real_vd) -> real_vd/1
  极坐标运动控制器/3(real_vq) -> real_vq/1
  [phi_2] -> 笛卡尔坐标系转极坐标系/2(phi_2)
  [phi_1] -> 笛卡尔坐标系转极坐标系/1(phi_1)
  Mux1/1 -> Reshape/1
  [L_0] -> Divide/2
  Constant1/1 -> Mux1/4  "M22"
  Reshape/1 -> [M]
  [M] -> 极坐标运动控制器/4(M)
  Constant/1 -> Mux1/3  "M12"
  Constant3/1 -> Mux1/2  "M21"
  Constant2/1 -> Divide/1
  Divide/1 -> Mux1/1  "M11"
  极坐标运动控制器/5(valid_tqd) -> valid_tqd/1
  [phi] -> 极坐标运动控制器/5(In5)
  Bus Selector/1 -> [phi_1]  "<phi_1>"
  Bus Selector/2 -> [phi_2]  "<phi_2>"
  phi/1 -> [phi], Bus Selector/1

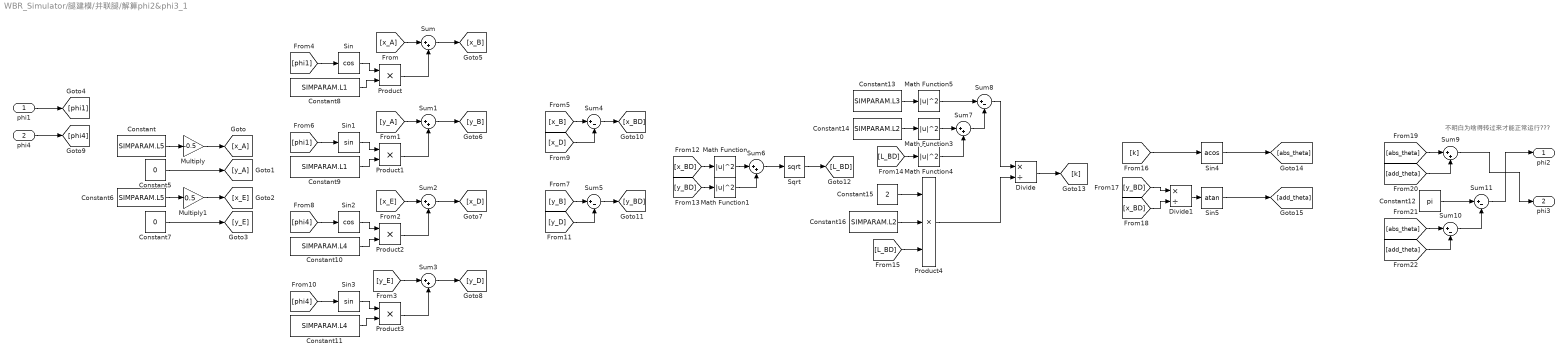
== system WBR_Simulator/腿建模/并联腿/解算phi2&phi3_1 ==
  note: 不明白为啥得转过来才能正常运行???
  phi1 : Inport
  phi4 : Inport  Port=2
  Constant : Constant  Value=SIMPARAM.L5
  Constant10 : Constant  Value=SIMPARAM.L4
  Constant11 : Constant  Value=SIMPARAM.L4
  Constant12 : Constant  Value=pi
  Constant13 : Constant  Value=SIMPARAM.L3
  Constant14 : Constant  Value=SIMPARAM.L2
  Constant15 : Constant  Value=2
  Constant16 : Constant  Value=SIMPARAM.L2
  Constant5 : Constant  Value=0
  Constant6 : Constant  Value=SIMPARAM.L5
  Constant7 : Constant  Value=0
  Constant8 : Constant  Value=SIMPARAM.L1
  Constant9 : Constant  Value=SIMPARAM.L1
  Divide : Product  Inputs=*/
  Divide1 : Product  Inputs=*/
  Math Function{,1,3..5} (5 alike) : Math  Operator=magnitude^2
  Multiply : Gain  Gain=-0.5
  Multiply1 : Gain  Gain=0.5
  Product{,1..3} (4 alike) : Product
  Product4 : Product  Inputs=3
  Sin : Trigonometry  Operator=cos
  Sin1 : Trigonometry
  Sin2 : Trigonometry  Operator=cos
  Sin3 : Trigonometry
  Sin4 : Trigonometry  Operator=acos
  Sin5 : Trigonometry  Operator=atan
  Sqrt : Sqrt
  Sum{,1..3,6..7,9} (7 alike) : Sum  Inputs=|++
  Sum{4..5,8,10..11} (5 alike) : Sum  Inputs=|+-
  phi2 : Outport
  phi3 : Outport  Port=2
  wires:
  Constant/1 -> Multiply/1
  Multiply/1 -> [x_A]
  Constant5/1 -> [y_A]
  Multiply1/1 -> [x_E]
  Constant6/1 -> Multiply1/1
  Constant7/1 -> [y_E]
  [x_A] -> Sum/1
  [phi1] -> Sin/1
  Sin/1 -> Product/1
  Product/1 -> Sum/2
  Constant8/1 -> Product/2
  phi1/1 -> [phi1]
  Constant9/1 -> Product1/2
  Product1/1 -> Sum1/2
  Sin1/1 -> Product1/1
  [y_A] -> Sum1/1
  [phi1] -> Sin1/1
  Constant10/1 -> Product2/2
  Product2/1 -> Sum2/2
  Sin2/1 -> Product2/1
  [x_E] -> Sum2/1
  [phi4] -> Sin2/1
  Constant11/1 -> Product3/2
  Product3/1 -> Sum3/2
  Sin3/1 -> Product3/1
  [y_E] -> Sum3/1
  [phi4] -> Sin3/1
  Sum/1 -> [x_B]
  Sum1/1 -> [y_B]
  Sum2/1 -> [x_D]
  Sum3/1 -> [y_D]
  phi4/1 -> [phi4]
  [x_B] -> Sum4/1
  [x_D] -> Sum4/2
  [y_B] -> Sum5/1
  [y_D] -> Sum5/2
  Sum4/1 -> [x_BD]
  Sum5/1 -> [y_BD]
  [x_BD] -> Math Function/1
  [y_BD] -> Math Function1/1
  Math Function/1 -> Sum6/1
  Math Function1/1 -> Sum6/2
  Sum6/1 -> Sqrt/1
  Sqrt/1 -> [L_BD]
  Constant14/1 -> Math Function3/1
  [L_BD] -> Math Function4/1
  Sum7/1 -> Sum8/2
  Math Function3/1 -> Sum7/1
  Math Function4/1 -> Sum7/2
  Sum8/1 -> Divide/1
  [L_BD] -> Product4/3
  Constant15/1 -> Product4/1
  Constant16/1 -> Product4/2
  Product4/1 -> Divide/2
  Divide/1 -> [k]
  [k] -> Sin4/1
  [y_BD] -> Divide1/1
  Sin5/1 -> [add_theta]
  [abs_theta] -> Sum9/1
  [add_theta] -> Sum9/2
  [x_BD] -> Divide1/2
  [abs_theta] -> Sum10/1
  [add_theta] -> Sum10/2
  Constant13/1 -> Math Function5/1
  Math Function5/1 -> Sum8/1
  Sum10/1 -> Sum11/2
  Constant12/1 -> Sum11/1
  Sin4/1 -> [abs_theta]
  Divide1/1 -> Sin5/1
  Sum11/1 -> phi2/1
  Sum9/1 -> phi3/1

== system WBR_Simulator/腿建模/并联腿/运动学解算验证(仅可证明旋转矩阵 ==
  R : Inport
  R_inv : Inport  Port=2
  Bus Creator1 : BusCreator  Inputs=2
  Bus Creator3 : BusCreator  Inputs=2
  Discrete Derivative : simulink/Discrete/Discrete Derivative  gainval=1.0  ICPrevScaledInput=0.0  OutMin=[]  OutMax=[]  OutDataType=fixdt(1, 16)  OutScaling=2^-10  DoSatur=off
  Discrete Derivative1 : simulink/Discrete/Discrete Derivative  gainval=1.0  ICPrevScaledInput=0.0  OutMin=[]  OutMax=[]  OutDataType=fixdt(1, 16)  OutScaling=2^-10  DoSatur=off
  Mux : Mux  Inputs=2
  Mux1 : Mux  Inputs=2
  PS-Simulink Converter{4..7} (4 alike) : nesl_utility/PS-Simulink Converter  PhysicalDomain=network_engine_domain  SubClassName=ps_output  LeftPortType=input  RightPortType=output  PseudoPeriodic=off  Frequencies=[]  VectorFormat=1-D array  Unit=inherit  AffineConversion=off
  Product : Product
  Product1 : Product  Multiplication=Matrix(*)
  Product2 : Product  Multiplication=Matrix(*)
  Transform Sensor : sm_lib/Frames and Transforms/Transform Sensor  MeasurementFrame=Base  RotationSequence=XYX  SenseAngle=off  SenseAxis=off  SenseQ=off  SenseR=off  SenseRotationSequence=off  SenseOmegaX=off  SenseOmegaY=off  SenseOmegaZ=off  SenseOmega=off  SenseQDot=off  SenseRDot=off  SenseRotationSequenceDot=off  SenseAlphaX=off  SenseAlphaY=off  SenseAlphaZ=off  SenseAlpha=off  SenseQDDot=off  SenseRDDot=off  SenseX=on  SenseY=off  SenseZ=on  SenseXYZ=off  SenseRad=off  SenseAzim=off  SenseDist=off  SenseInc=off  SenseXDot=on  SenseYDot=off  SenseZDot=on  SenseXYZDot=off  SenseRadDot=off  SenseAzimDot=off  SenseDistDot=off  SenseIncDot=off  SenseXDDot=off  SenseYDDot=off  SenseZDDot=off  SenseXYZDDot=off  SenseRadDDot=off  SenseAzimDDot=off  SenseDistDDot=off  SenseIncDDot=off
  Zero-Order Hold{,1..3} (4 alike) : ZeroOrderHold  SampleTime=0.001
  笛卡尔转极坐标 : Subsystem
  五连杆末端坐标 : PMIOPort  Side=Right
  基坐标 : PMIOPort  Port=2  Side=Left
  wires:
  Discrete Derivative/1 -> Product/1
  Product1/1 -> ?  "代算C点正交坐标速度"
  [R] -> Product2/1
  Discrete Derivative1/1 -> Mux/2, Bus Creator1/2  "vd"
  笛卡尔转极坐标/2(L_0) -> Discrete Derivative1/1, Product/2
  Mux/1 -> Product1/2
  笛卡尔转极坐标/1(phi_0) -> Discrete Derivative/1
  [R_inv] -> Product1/1
  Product/1 -> Mux/1, Bus Creator1/1  "vq"
  PS-Simulink Converter5/1 -> Zero-Order Hold1/1
  Bus Creator1/1 -> ?  "真实C点极坐标速度"
  PS-Simulink Converter4/1 -> Zero-Order Hold/1
  Mux1/1 -> Product2/2
  Product2/1 -> ?  "代算C点极坐标速度"
  Bus Creator3/1 -> ?  "真实C点正交坐标速度"
  R/1 -> [R]
  R_inv/1 -> [R_inv]
  Zero-Order Hold/1 -> 笛卡尔转极坐标/1(x)
  Zero-Order Hold1/1 -> 笛卡尔转极坐标/2(z)
  Zero-Order Hold3/1 -> Mux1/2, Bus Creator3/2
  PS-Simulink Converter7/1 -> Zero-Order Hold3/1  "vz"
  Zero-Order Hold2/1 -> Mux1/1, Bus Creator3/1
  PS-Simulink Converter6/1 -> Zero-Order Hold2/1  "vx"
  connections:
  PS-Simulink Converter5/LConn1 -- Transform Sensor/RConn3
  PS-Simulink Converter4/LConn1 -- Transform Sensor/RConn2
  Transform Sensor/RConn1 -- 五连杆末端坐标/RConn1
  基坐标/RConn1 -- Transform Sensor/LConn1
  PS-Simulink Converter6/LConn1 -- Transform Sensor/RConn4
  PS-Simulink Converter7/LConn1 -- Transform Sensor/RConn5

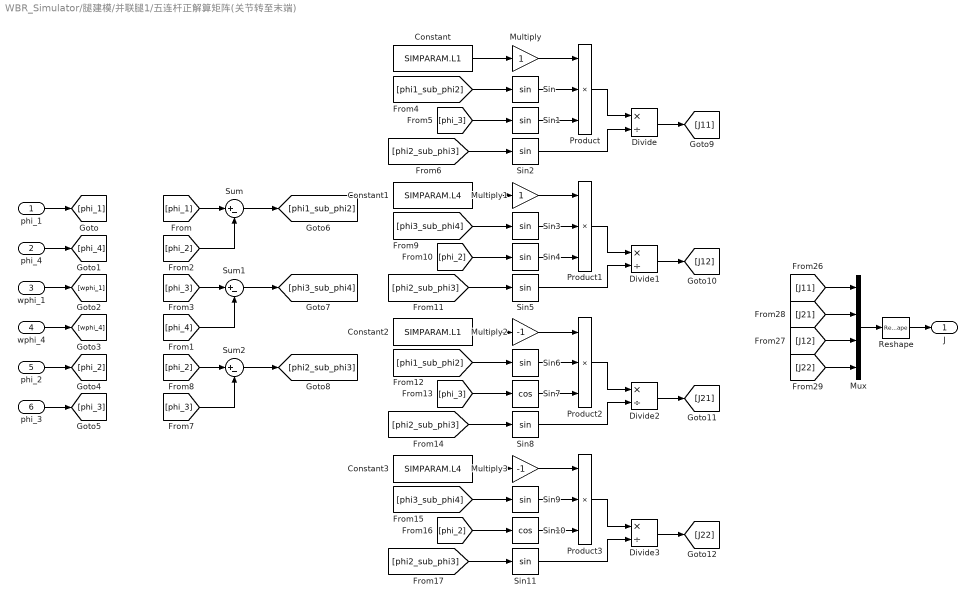
== system WBR_Simulator/腿建模/并联腿1/五连杆正解算矩阵(关节转至末端) ==
  phi_1 : Inport
  phi_4 : Inport  Port=2
  wphi_1 : Inport  Port=3
  wphi_4 : Inport  Port=4
  phi_2 : Inport  Port=5
  phi_3 : Inport  Port=6
  Constant : Constant  Value=SIMPARAM.L1
  Constant1 : Constant  Value=SIMPARAM.L4
  Constant2 : Constant  Value=SIMPARAM.L1
  Constant3 : Constant  Value=SIMPARAM.L4
  Divide{,1..3} (4 alike) : Product  Inputs=*/
  Multiply : Gain
  Multiply1 : Gain
  Multiply2 : Gain  Gain=-1
  Multiply3 : Gain  Gain=-1
  Mux : Mux
  Product{,1..3} (4 alike) : Product  Inputs=3
  Reshape : Reshape  OutputDimensionality=Customize  OutputDimensions=[2,2]
  Sin{,1..6,8..9,11} (10 alike) : Trigonometry
  Sin10 : Trigonometry  Operator=cos
  Sin7 : Trigonometry  Operator=cos
  Sum : Sum  Inputs=|+-
  Sum1 : Sum  Inputs=|+-
  Sum2 : Sum  Inputs=|+-
  J : Outport
  wires:
  phi_1/1 -> [phi_1]
  phi_4/1 -> [phi_4]
  wphi_1/1 -> [wphi_1]
  wphi_4/1 -> [wphi_4]
  phi_2/1 -> [phi_2]
  phi_3/1 -> [phi_3]
  [phi_1] -> Sum/1
  [phi_2] -> Sum/2
  Sum/1 -> [phi1_sub_phi2]
  Sum1/1 -> [phi3_sub_phi4]
  [phi_3] -> Sum1/1
  [phi_4] -> Sum1/2
  [phi1_sub_phi2] -> Sin/1
  Sin/1 -> Product/2
  Constant/1 -> Multiply/1
  Multiply/1 -> Product/1
  [phi_3] -> Sin1/1
  Sin1/1 -> Product/3
  Product/1 -> Divide/1
  [phi2_sub_phi3] -> Sin2/1
  Sin2/1 -> Divide/2
  [phi_3] -> Sum2/2
  [phi_2] -> Sum2/1
  Sum2/1 -> [phi2_sub_phi3]
  Divide/1 -> [J11]
  Product1/1 -> Divide1/1
  Constant1/1 -> Multiply1/1
  [phi3_sub_phi4] -> Sin3/1
  Divide1/1 -> [J12]
  Sin5/1 -> Divide1/2
  [phi_2] -> Sin4/1
  Multiply1/1 -> Product1/1
  Sin4/1 -> Product1/3
  [phi2_sub_phi3] -> Sin5/1
  Sin3/1 -> Product1/2
  Product2/1 -> Divide2/1
  Constant2/1 -> Multiply2/1
  [phi1_sub_phi2] -> Sin6/1
  Divide2/1 -> [J21]
  Sin8/1 -> Divide2/2
  [phi_3] -> Sin7/1
  Multiply2/1 -> Product2/1
  Sin7/1 -> Product2/3
  [phi2_sub_phi3] -> Sin8/1
  Sin6/1 -> Product2/2
  Product3/1 -> Divide3/1
  Constant3/1 -> Multiply3/1
  [phi3_sub_phi4] -> Sin9/1
  Divide3/1 -> [J22]
  Sin11/1 -> Divide3/2
  [phi_2] -> Sin10/1
  Multiply3/1 -> Product3/1
  Sin10/1 -> Product3/3
  [phi2_sub_phi3] -> Sin11/1
  Sin9/1 -> Product3/2
  [J11] -> Mux/1
  [J22] -> Mux/4
  Mux/1 -> Reshape/1
  Reshape/1 -> J/1
  [J21] -> Mux/2
  [J12] -> Mux/3

== system WBR_Simulator/腿建模/并联腿1/腿末端控制器 ==
  phi : Inport
  wphi_1 : Inport  Port=2
  wphi_4 : Inport  Port=3
  set_tq : Inport  Port=4
  set_fd : Inport  Port=5
  J : Inport  Port=6
  Bus Selector : BusSelector  OutputSignals=phi_1,phi_2
  Constant : Constant  Value=0
  Constant1 : Constant
  Constant2 : Constant
  Constant3 : Constant  Value=0
  Divide : Product  Inputs=*/
  Mux : Mux  Inputs=2
  Mux1 : Mux
  Product : Product  Inputs=/  Multiplication=Matrix(*)
  Product8 : Product  Multiplication=Matrix(*)
  Reshape : Reshape  OutputDimensionality=Customize  OutputDimensions=[2,2]
  极坐标运动控制器 : Subsystem
  笛卡尔坐标系转极坐标系 : Subsystem
  torque_1 : Outport
  torque_4 : Outport  Port=2
  R : Outport  Port=3
  R_inv : Outport  Port=4
  phi_0 : Outport  Port=5
  L_0 : Outport  Port=6
  real_vq : Outport  Port=7
  real_vd : Outport  Port=8
  valid_tqd : Outport  Port=9
  wires:
  J/1 -> [J]
  wphi_1/1 -> [wphi_1]
  wphi_4/1 -> [wphi_4]
  Product8/1 -> [real_vxy]
  [wphi_4] -> Mux/2
  [J] -> Product8/1
  Mux/1 -> Product8/2
  [wphi_1] -> Mux/1
  [real_vxy] -> 极坐标运动控制器/1(real_vxy)
  [R] -> 极坐标运动控制器/2(R)
  [J] -> 极坐标运动控制器/3(J)
  笛卡尔坐标系转极坐标系/1(R) -> [R], R/1, Product/1
  Product/1 -> R_inv/1
  极坐标运动控制器/2(torque_4) -> torque_4/1
  极坐标运动控制器/1(torque_1) -> torque_1/1
  笛卡尔坐标系转极坐标系/3(L_0) -> [L_0], L_0/1
  笛卡尔坐标系转极坐标系/2(phi_0) -> phi_0/1
  set_tq/1 -> 极坐标运动控制器/6(set_tq)
  set_fd/1 -> 极坐标运动控制器/7(set_fd)
  极坐标运动控制器/4(real_vd) -> real_vd/1
  极坐标运动控制器/3(real_vq) -> real_vq/1
  [phi_2] -> 笛卡尔坐标系转极坐标系/2(phi_2)
  [phi_1] -> 笛卡尔坐标系转极坐标系/1(phi_1)
  Mux1/1 -> Reshape/1
  [L_0] -> Divide/2
  Constant1/1 -> Mux1/4  "M22"
  Reshape/1 -> [M]
  [M] -> 极坐标运动控制器/4(M)
  Constant/1 -> Mux1/3  "M12"
  Constant3/1 -> Mux1/2  "M21"
  Constant2/1 -> Divide/1
  Divide/1 -> Mux1/1  "M11"
  极坐标运动控制器/5(valid_tqd) -> valid_tqd/1
  [phi] -> 极坐标运动控制器/5(In5)
  Bus Selector/1 -> [phi_1]  "<phi_1>"
  Bus Selector/2 -> [phi_2]  "<phi_2>"
  phi/1 -> [phi], Bus Selector/1

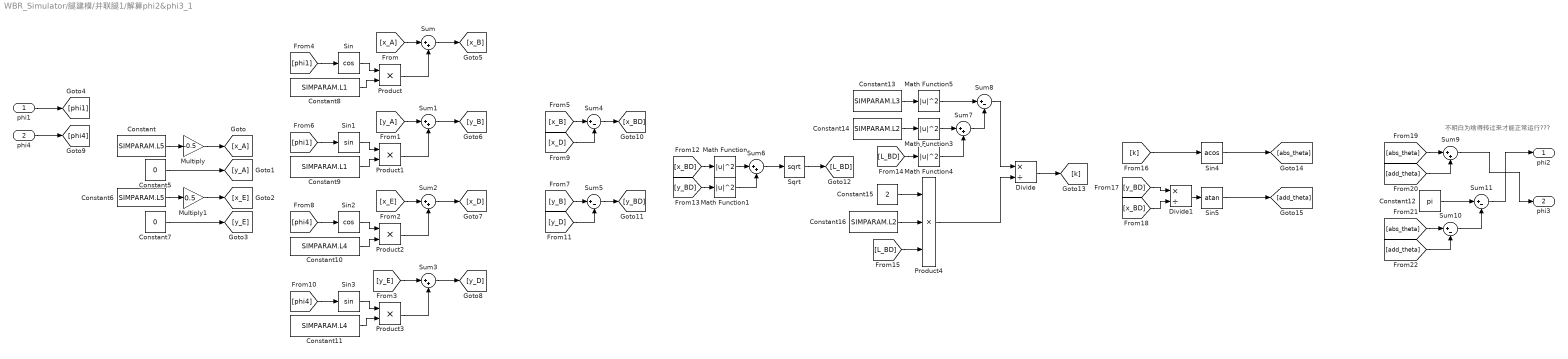
== system WBR_Simulator/腿建模/并联腿1/解算phi2&phi3_1 ==
  note: 不明白为啥得转过来才能正常运行???
  phi1 : Inport
  phi4 : Inport  Port=2
  Constant : Constant  Value=SIMPARAM.L5
  Constant10 : Constant  Value=SIMPARAM.L4
  Constant11 : Constant  Value=SIMPARAM.L4
  Constant12 : Constant  Value=pi
  Constant13 : Constant  Value=SIMPARAM.L3
  Constant14 : Constant  Value=SIMPARAM.L2
  Constant15 : Constant  Value=2
  Constant16 : Constant  Value=SIMPARAM.L2
  Constant5 : Constant  Value=0
  Constant6 : Constant  Value=SIMPARAM.L5
  Constant7 : Constant  Value=0
  Constant8 : Constant  Value=SIMPARAM.L1
  Constant9 : Constant  Value=SIMPARAM.L1
  Divide : Product  Inputs=*/
  Divide1 : Product  Inputs=*/
  Math Function{,1,3..5} (5 alike) : Math  Operator=magnitude^2
  Multiply : Gain  Gain=-0.5
  Multiply1 : Gain  Gain=0.5
  Product{,1..3} (4 alike) : Product
  Product4 : Product  Inputs=3
  Sin : Trigonometry  Operator=cos
  Sin1 : Trigonometry
  Sin2 : Trigonometry  Operator=cos
  Sin3 : Trigonometry
  Sin4 : Trigonometry  Operator=acos
  Sin5 : Trigonometry  Operator=atan
  Sqrt : Sqrt
  Sum{,1..3,6..7,9} (7 alike) : Sum  Inputs=|++
  Sum{4..5,8,10..11} (5 alike) : Sum  Inputs=|+-
  phi2 : Outport
  phi3 : Outport  Port=2
  wires:
  Constant/1 -> Multiply/1
  Multiply/1 -> [x_A]
  Constant5/1 -> [y_A]
  Multiply1/1 -> [x_E]
  Constant6/1 -> Multiply1/1
  Constant7/1 -> [y_E]
  [x_A] -> Sum/1
  [phi1] -> Sin/1
  Sin/1 -> Product/1
  Product/1 -> Sum/2
  Constant8/1 -> Product/2
  phi1/1 -> [phi1]
  Constant9/1 -> Product1/2
  Product1/1 -> Sum1/2
  Sin1/1 -> Product1/1
  [y_A] -> Sum1/1
  [phi1] -> Sin1/1
  Constant10/1 -> Product2/2
  Product2/1 -> Sum2/2
  Sin2/1 -> Product2/1
  [x_E] -> Sum2/1
  [phi4] -> Sin2/1
  Constant11/1 -> Product3/2
  Product3/1 -> Sum3/2
  Sin3/1 -> Product3/1
  [y_E] -> Sum3/1
  [phi4] -> Sin3/1
  Sum/1 -> [x_B]
  Sum1/1 -> [y_B]
  Sum2/1 -> [x_D]
  Sum3/1 -> [y_D]
  phi4/1 -> [phi4]
  [x_B] -> Sum4/1
  [x_D] -> Sum4/2
  [y_B] -> Sum5/1
  [y_D] -> Sum5/2
  Sum4/1 -> [x_BD]
  Sum5/1 -> [y_BD]
  [x_BD] -> Math Function/1
  [y_BD] -> Math Function1/1
  Math Function/1 -> Sum6/1
  Math Function1/1 -> Sum6/2
  Sum6/1 -> Sqrt/1
  Sqrt/1 -> [L_BD]
  Constant14/1 -> Math Function3/1
  [L_BD] -> Math Function4/1
  Sum7/1 -> Sum8/2
  Math Function3/1 -> Sum7/1
  Math Function4/1 -> Sum7/2
  Sum8/1 -> Divide/1
  [L_BD] -> Product4/3
  Constant15/1 -> Product4/1
  Constant16/1 -> Product4/2
  Product4/1 -> Divide/2
  Divide/1 -> [k]
  [k] -> Sin4/1
  [y_BD] -> Divide1/1
  Sin5/1 -> [add_theta]
  [abs_theta] -> Sum9/1
  [add_theta] -> Sum9/2
  [x_BD] -> Divide1/2
  [abs_theta] -> Sum10/1
  [add_theta] -> Sum10/2
  Constant13/1 -> Math Function5/1
  Math Function5/1 -> Sum8/1
  Sum10/1 -> Sum11/2
  Constant12/1 -> Sum11/1
  Sin4/1 -> [abs_theta]
  Divide1/1 -> Sin5/1
  Sum11/1 -> phi2/1
  Sum9/1 -> phi3/1
